simulink model "student_model_ref_2024a"  (R2024a)
settings: Solver=VariableStepAuto  StartTime=0.0  StopTime=t_sim  RelTol=1e-5  EnableMultiTasking=on
values from neighbouring files (symbols this model uses):
  A = [0 1; -wn_model^2 -2*zeta_model*wn_model]    [student_lab3_model_ref.m]
  Ap = [0 1; -wn^2 -2*zeta*wn]    [student_lab3_model_ref.m]
  B = [0; 1]    [student_lab3_model_ref.m]
  Bp = [0; 1]    [student_lab3_model_ref.m]
  C = eye(2)    [student_lab3_model_ref.m]
  Cp = eye(2)    [student_lab3_model_ref.m]
  D = [0;0]    [student_lab3_model_ref.m]
  Dp = [0;0]    [student_lab3_model_ref.m]
  step1 = v_step    (= 0.2)    [student_lab3_model_ref.m]
  step2 = -v_step    (= -0.2)    [student_lab3_model_ref.m]
  t_off = 5    [student_lab3_model_ref.m]
  t_on = 1    [student_lab3_model_ref.m]
undefined symbols (not defined in the file or in its folder): student_model_ref_controller
settings Model: Creator=Kelvin  LastModifiedBy=wbarclay6
settings SolverCC: AlgebraicLoopSolver=TrustRegion
settings DataIOCC: LimitDataPoints=on  SaveFormat=Array  SignalLoggingSaveFormat=ModelDataLogs  ReturnWorkspaceOutputs=off
settings OptimizationCC: ExpressionDepthLimit=2147483647  LifeSpan=inf
settings DebuggingCC: UnderspecifiedInitializationDetection=Classic  MergeDetectMultiDrivingBlocksExec=none  SolverPrmCheckMsg=warning  FcnCallInpInsideContextMsg=warning  UnconnectedInputMsg=warning  UnconnectedOutputMsg=warning  UnconnectedLineMsg=warning  StateNameClashWarn=warning  SFUnexpectedBacktrackingDiag=warning  SFNoUnconditionalDefaultTransitionDiag=warning  SFExecutionAtInitializationDiag=none  ArithmeticOperatorsInVariantConditions=warning
settings HardwareCC: ProdBitPerPointer=32  ProdBitPerSizeT=32  ProdBitPerPtrDiffT=32  ProdLargestAtomicFloat=None  ProdIntDivRoundTo=Undefined  ProdEndianess=Unspecified  ProdWordSize=32  ProdHWDeviceType=32-bit Generic
settings ModelReferenceCC: EnableRefExpFcnMdlSchedulingChecks=on  PropagateSignalLabelsOutOfModel=off
settings SFSimCC: SimUseLocalCustomCode=off  CustomCodeUndefinedFunction=UseInterfaceOnly
settings RTWCC: RTWUseLocalCustomCode=off  GPUComputeCapability=3.5  DLArmComputeVersion=19.05
settings CodeAppCC: StateflowObjectComments=on
settings GRTTargetCC: TargetLangStandard=C89/C90 (ANSI)  CombineOutputUpdateFcns=off  GRTInterface=on
settings ConfigComp: CovMetricSettings=dw  CovSaveCumulativeToWorkspaceVar=on  CovSaveSingleToWorkspaceVar=on  CovExternalEMLEnable=off

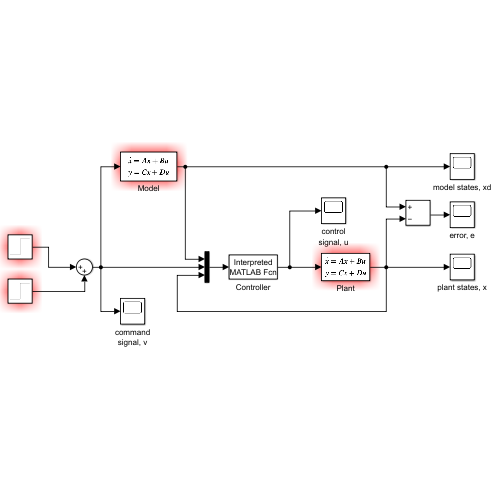
[thumbnail: Simulink's stored preview of the top-level diagram]
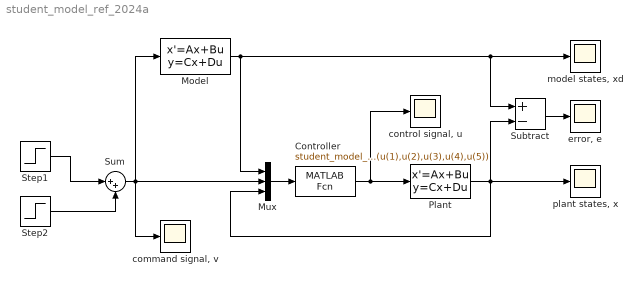
== system student_model_ref_2024a ==
  Controller : MATLABFcn  MATLABFcn=student_model_ref_controller(u(1),u(2),u(3),u(4),u(5))
  Model : StateSpace  A=A  B=B  C=C  D=D  InitialCondition=0
  Mux : Mux  Inputs=3
  Plant : StateSpace  A=Ap  B=Bp  C=Cp  D=Dp  InitialCondition=0
  Step1 : Step  Time=t_on  After=step1  SampleTime=0  ZeroCross=off
  Step2 : Step  Time=t_off  After=step2  SampleTime=0  ZeroCross=off
  Subtract : Sum  Inputs=+-
  Sum : Sum  Inputs=|++
  "command signal, v" : Scope
  "control signal, u" : Scope
  "error, e" : Scope
  "model states, xd" : Scope
  "plant states, x" : Scope
  wires:
  Sum/1 -> Mux/2, "command signal, v"/1, Model/1
  Mux/1 -> Controller/1
  Controller/1 -> "control signal, u"/1, Plant/1
  Plant/1 -> Mux/3, "plant states, x"/1, Subtract/2
  Model/1 -> Mux/1, Subtract/1, "model states, xd"/1
  Subtract/1 -> "error, e"/1
  Step1/1 -> Sum/1
  Step2/1 -> Sum/2
